simulink model "mcb_pmsm_foc_sensorless_f28069MLaunchPad"  (R2024a)
settings: Solver=FixedStepDiscrete  StartTime=0.0  StopTime=8  RelTol=1e-3  EnableMultiTasking=on
InitFcn:
  | mcb_pmsm_foc_sensorless_f28069MLaunchPad_datascript;
undefined symbols (not defined in the file): acceleration, Down, GPTRIP1SEL, GPTRIP2SEL, inverter, MAX_OL_NEG_SPD, MAX_OL_POS_SPD, MAX_OL_VD_LIMIT, MIN_CL_NEG_SPD, MIN_CL_POS_SPD, MIN_OL_VD_LIMIT, one_sec_tick, PI_params, pmsm, PU_System, RAMP_STEP_SIZE, target, Ts, Ts_motor, Ts_simulink, Ts_speed, two_sec_tick, TZ1, TZ2, Up
libraries: mcbcontrolslib x16, c2802xlib x5, simulink x4, c280xlib x4, slpidlib x3, mcbpositiondecoderlib x3, c2806xlib x3, mcbsensorlessestimatorlib x2, svdschedulerlib x2, mcbplantlib x1, autolibpmsmexterior x1
(part 2 of 3)

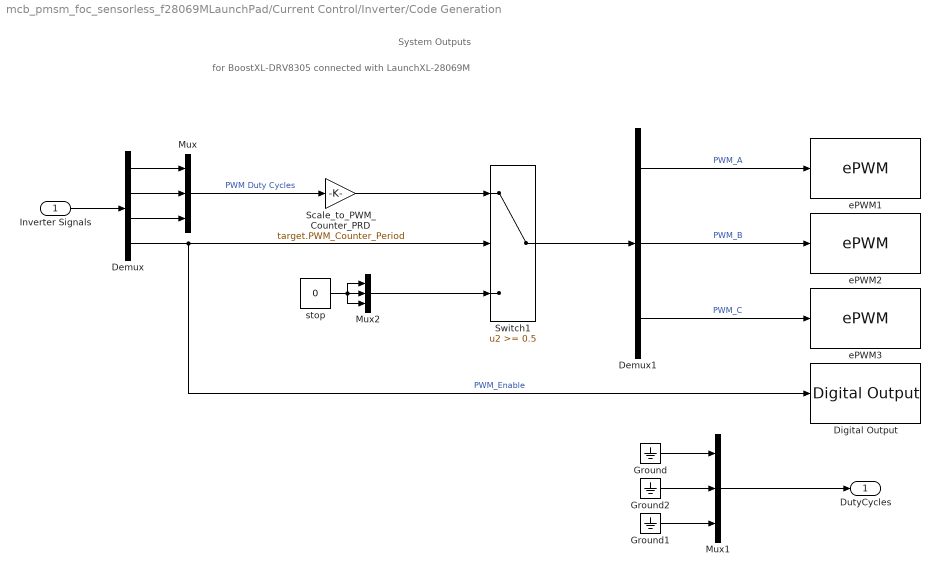
== system mcb_pmsm_foc_sensorless_f28069MLaunchPad/Current Control/Inverter/Code Generation ==
  note: for BoostXL-DRV8305 connected with LaunchXL-28069M
  note: System Outputs
  Inverter Signals : Inport
  Demux : Demux
  Demux1 : Demux  Outputs=3
  Digital Output : c2806xlib/Digital Output  GPIO_Number=GPIO50~GPIO55  GPIO_Bit0=off  GPIO_BIT0_Toggle=off  GPIO_Bit1=off  GPIO_BIT1_Toggle=off  GPIO_Bit2=on  GPIO_BIT2_Toggle=off  GPIO_Bit3=off  GPIO_BIT3_Toggle=off  GPIO_Bit4=off  GPIO_BIT4_Toggle=off  GPIO_Bit5=off  GPIO_BIT5_Toggle=off  GPIO_Bit6=off  GPIO_BIT6_Toggle=off  GPIO_Bit7=off  GPIO_BIT7_Toggle=off
  Ground : Ground
  Ground1 : Ground
  Ground2 : Ground
  Mux : Mux  Inputs=3
  Mux1 : Mux  Inputs=3
  Mux2 : Mux  Inputs=3
  Scale_to_PWM_Counter_PRD : Gain  Gain=target.PWM_Counter_Period  OutDataTypeStr=uint16  RndMeth=Simplest
  Switch1 : Switch  Threshold=0.5  SaturateOnIntegerOverflow=off  InputSameDT=off
  ePWM1 : c2802xlib/ePWM  PwmType=C2000  useModule=ePWM1  ePWMxLINKTBPRD=Not Linked  periodUnits=Clock cycles  timerSource=Specify via dialog  timerPeriod_clk=target.PWM_Counter_Period  timerPeriod_sec=64000  tbshadow=Counter equals to zero  countingMode=Up-Down  phaseActiveEnable=Disable  phaseDirection=Count down after sync  phaseActive=0  synchronizationEnable=off  dcaevt1Sync=off  dcbevt1Sync=off  synchronizationOption=Counter equals to zero (CTR=Zero)  dcbevt1SyncOut=off  dcaevt1SyncOut=off  cmpdSyncOut=off  cmpcSyncOut=off  cmpbSyncOut=off  zeroSyncOut=on  swfSyncOut=off  perSynchronizationOption=Counter equals to period (CTR=PRD)  clockPrescale=1  HSclockPrescale=1  enswap=off  ePWMxAStatus=on  ePWMxAactionLogic1=Do nothing  ePWMxAactionLogic2=Do nothing  ePWMxAactionLogic3=Clear  ePWMxAactionLogic4=Set  ePWMxAactionLogic5=Do nothing  ePWMxAactionLogic6=Do nothing  ePWMxACSFenable=off  ePWMxACSFvalue=Forcing disable  ePWMxASFreload=Zero  ePWMxBStatus=off  ePWMxBactionLogic1=Do nothing  ePWMxBactionLogic2=Set  ePWMxBactionLogic3=Do nothing  ePWMxBactionLogic4=Do nothing  ePWMxBactionLogic5=Clear  ePWMxBactionLogic6=Do nothing  ePWMxBCSFenable=off  ePWMxBCSFvalue=Forcing disable  ePWMxBSFreload=Zero  ePWNxBOutWay=off  ePWMxLINKCMPA=Not Linked  CMPAUnits=Clock cycles  CMPASource=Input port  CMPAValue_per=32000  CMPAValue_clk=floor(target.PWM_Counter_Period/2+1)  enCMPAshadow=Counter equals to zero (CTR=Zero)  ePWMxLINKCMPB=Not Linked  CMPBUnits=Clock cycles  CMPBSource=Specify via dialog  CMPBValue_per=50  CMPBValue_clk=floor(target.PWM_Counter_Period/2+1)  enCMPBshadow=Counter equals to zero (CTR=Zero)  ePWMxLINKCMPC=Not Linked  CMPCUnits=Clock cycles  CMPCSource=Specify via dialog  CMPCValue_per=50  CMPCValue_clk=32000  enCMPCshadow=Counter equals to zero (CTR=Zero)  ePWMxLINKCMPD=Not Linked  CMPDUnits=Clock cycles  CMPDSource=Specify via dialog  CMPDValue_per=50  CMPDValue_clk=32000  enCMPDshadow=Counter equals to zero (CTR=Zero)  enableDBePWMxA=on  enableDBePWMxB=on  enhalfcycle=off  DBpolarity=Active high complementary (AHC)  DBedgeDelay=Positive  DBSource_ePWMxA=ePWMxA  DBSource_ePWMxB=ePWMxA  DBPeriodUnits=Clock cycles  DBperiodSource=Specify via dialog  REDperiod=15  FEDperiod=15  REDperiod_sec=0  FEDperiod_sec=0  LoadModeDBRED=Immediate without using shadow  LoadModeDBFED=Immediate without using shadow  adcstartModuleA=on  adcrequestEventA=First event  adcstartEventA=Counter equals to period (CTR=PRD)  adcstartEventA_type2=Digital Compare Module A Event 1 start of conversion (DCAEVT1.soc)  adcstartModuleB=off  adcrequestEventB=First event  adcstartEventB=Counter equals to zero (CTR=Zero)  adcstartEventB_type2=Counter equals to zero (CTR=Zero)  intEn=off  intPrd=First event  intSel=Counter equals to zero (CTR=Zero)  intSel_type2=Counter equals to zero (CTR=Zero)  hrpe=off  enHRPWM=off  HRPWM_LoadMode=Counter equals to period (CTR=PRD)  HRPWM_CTLMode=Duty or Period control mode  HRPWM_EDGMode=Both edge  hrpeb=off  enHRPWMB=off  HRPWM_LoadModeB=Counter equals to zero (CTR=ZERO)  HRPWM_CTLModeB=Duty or Period control mode  HRPWM_EDGModeB=Both edge  enHRDBRED=off  enHRDBFED=off  enSFO=on  enautoconv=on  chopperEnable=off  chopperFrequency=1  chopperFirstwidth=1  chopperDuty=12.5%  tripZonesource=Specify via dialog  tzselOSHT1=off  tzselOSHT2=off  tzselOSHT3=off  tzselOSHT4=off  tzselOSHT5=off  tzselOSHT6=off  tzselOSHDCAEV1=off  tzselOSHDCBEV1=off  tzselCBC1=off  tzselCBC2=off  tzselCBC3=off  tzselCBC4=off  tzselCBC5=off  tzselCBC6=off  tzselCBCDCAEV2=off  tzselCBCDCBEV2=off  enTzOstIntr=off  enTzCbcIntr=off  enTzDCAEVT1Intr=off  enTzDCAEVT2Intr=off  enTzDCBEVT1Intr=off  enTzDCBEVT2Intr=off  tzclrCBCLatch=Counter equals to zero (CTR=Zero)  ePWMxAforced=No action  ePWMxBforced=No action  DCAEVT1forced=No action  DCBEVT1forced=No action  DCAEVT2forced=No action  DCBEVT2forced=No action  dcah=Trip Zone 1 input (TZ1)  dcal=Trip Zone 2 input (TZ2)  dcbh=Trip Zone 1 input (TZ1)  dcbl=Trip Zone 2 input (TZ2)  dcah_type2=GPTRIP1SEL/(TZ1)  dcal_type2=GPTRIP2SEL/(TZ2)  dcbh_type2=GPTRIP1SEL/(TZ1)  dcbl_type2=GPTRIP2SEL/(TZ2)  gendcaevt1=Event disabled  gendcaevt2=Event disabled  gendcbevt1=Event disabled  gendcbevt2=Event disabled  dcaevt1src=DCAEVT1 with sync  dcaevt2src=DCAEVT2 with sync  dcbevt1src=DCBEVT1 with sync  dcbevt2src=DCBEVT2 with sync  pulsesel=Counter equals to zero (CTR=Zero)  blankinv=off  blankoffset=0  blankwidth=0  evsrcsel=Filtered version of DCAEVT1 (DCAEVT1FILT)  encape=off
  ePWM2 : c2802xlib/ePWM  PwmType=C2000  useModule=ePWM2  ePWMxLINKTBPRD=Not Linked  periodUnits=Clock cycles  timerSource=Specify via dialog  timerPeriod_clk=target.PWM_Counter_Period  timerPeriod_sec=64000  tbshadow=Counter equals to zero  countingMode=Up-Down  phaseActiveEnable=Set counter to phase value specified via dialog  phaseDirection=Count up after sync  phaseActive=0  synchronizationEnable=off  dcaevt1Sync=off  dcbevt1Sync=off  synchronizationOption=Pass through (EPWMxSYNCI or SWFSYNC)  dcbevt1SyncOut=off  dcaevt1SyncOut=off  cmpdSyncOut=off  cmpcSyncOut=off  cmpbSyncOut=off  zeroSyncOut=off  swfSyncOut=on  perSynchronizationOption=Counter equals to period (CTR=PRD)  clockPrescale=1  HSclockPrescale=1  enswap=off  ePWMxAStatus=on  ePWMxAactionLogic1=Do nothing  ePWMxAactionLogic2=Do nothing  ePWMxAactionLogic3=Clear  ePWMxAactionLogic4=Set  ePWMxAactionLogic5=Do nothing  ePWMxAactionLogic6=Do nothing  ePWMxACSFenable=off  ePWMxACSFvalue=Forcing disable  ePWMxASFreload=Zero  ePWMxBStatus=off  ePWMxBactionLogic1=Do nothing  ePWMxBactionLogic2=Set  ePWMxBactionLogic3=Do nothing  ePWMxBactionLogic4=Do nothing  ePWMxBactionLogic5=Clear  ePWMxBactionLogic6=Do nothing  ePWMxBCSFenable=off  ePWMxBCSFvalue=Forcing disable  ePWMxBSFreload=Zero  ePWNxBOutWay=off  ePWMxLINKCMPA=Not Linked  CMPAUnits=Clock cycles  CMPASource=Input port  CMPAValue_per=32000  CMPAValue_clk=floor(target.PWM_Counter_Period/2+1)  enCMPAshadow=Counter equals to zero (CTR=Zero)  ePWMxLINKCMPB=Not Linked  CMPBUnits=Clock cycles  CMPBSource=Specify via dialog  CMPBValue_per=50  CMPBValue_clk=floor(target.PWM_Counter_Period/2+1)  enCMPBshadow=Counter equals to zero (CTR=Zero)  ePWMxLINKCMPC=Not Linked  CMPCUnits=Clock cycles  CMPCSource=Specify via dialog  CMPCValue_per=50  CMPCValue_clk=32000  enCMPCshadow=Counter equals to zero (CTR=Zero)  ePWMxLINKCMPD=Not Linked  CMPDUnits=Clock cycles  CMPDSource=Specify via dialog  CMPDValue_per=50  CMPDValue_clk=32000  enCMPDshadow=Counter equals to zero (CTR=Zero)  enableDBePWMxA=on  enableDBePWMxB=on  enhalfcycle=off  DBpolarity=Active high complementary (AHC)  DBedgeDelay=Positive  DBSource_ePWMxA=ePWMxA  DBSource_ePWMxB=ePWMxA  DBPeriodUnits=Clock cycles  DBperiodSource=Specify via dialog  REDperiod=15  FEDperiod=15  REDperiod_sec=0  FEDperiod_sec=0  LoadModeDBRED=Immediate without using shadow  LoadModeDBFED=Immediate without using shadow  adcstartModuleA=off  adcrequestEventA=First event  adcstartEventA=Digital Compare Module A Event 1 start of conversion (DCAEVT1.soc)  adcstartEventA_type2=Digital Compare Module A Event 1 start of conversion (DCAEVT1.soc)  adcstartModuleB=off  adcrequestEventB=First event  adcstartEventB=Counter equals to zero (CTR=Zero)  adcstartEventB_type2=Counter equals to zero (CTR=Zero)  intEn=off  intPrd=First event  intSel=Counter equals to zero (CTR=Zero)  intSel_type2=Counter equals to zero (CTR=Zero)  hrpe=off  enHRPWM=off  HRPWM_LoadMode=Counter equals to period (CTR=PRD)  HRPWM_CTLMode=Duty or Period control mode  HRPWM_EDGMode=Both edge  hrpeb=off  enHRPWMB=off  HRPWM_LoadModeB=Counter equals to zero (CTR=ZERO)  HRPWM_CTLModeB=Duty or Period control mode  HRPWM_EDGModeB=Both edge  enHRDBRED=off  enHRDBFED=off  enSFO=on  enautoconv=on  chopperEnable=off  chopperFrequency=1  chopperFirstwidth=1  chopperDuty=12.5%  tripZonesource=Specify via dialog  tzselOSHT1=off  tzselOSHT2=off  tzselOSHT3=off  tzselOSHT4=off  tzselOSHT5=off  tzselOSHT6=off  tzselOSHDCAEV1=off  tzselOSHDCBEV1=off  tzselCBC1=off  tzselCBC2=off  tzselCBC3=off  tzselCBC4=off  tzselCBC5=off  tzselCBC6=off  tzselCBCDCAEV2=off  tzselCBCDCBEV2=off  enTzOstIntr=off  enTzCbcIntr=off  enTzDCAEVT1Intr=off  enTzDCAEVT2Intr=off  enTzDCBEVT1Intr=off  enTzDCBEVT2Intr=off  tzclrCBCLatch=Counter equals to zero (CTR=Zero)  ePWMxAforced=No action  ePWMxBforced=No action  DCAEVT1forced=No action  DCBEVT1forced=No action  DCAEVT2forced=No action  DCBEVT2forced=No action  dcah=Trip Zone 1 input (TZ1)  dcal=Trip Zone 2 input (TZ2)  dcbh=Trip Zone 1 input (TZ1)  dcbl=Trip Zone 2 input (TZ2)  dcah_type2=GPTRIP1SEL/(TZ1)  dcal_type2=GPTRIP2SEL/(TZ2)  dcbh_type2=GPTRIP1SEL/(TZ1)  dcbl_type2=GPTRIP2SEL/(TZ2)  gendcaevt1=Event disabled  gendcaevt2=Event disabled  gendcbevt1=Event disabled  gendcbevt2=Event disabled  dcaevt1src=DCAEVT1 with sync  dcaevt2src=DCAEVT2 with sync  dcbevt1src=DCBEVT1 with sync  dcbevt2src=DCBEVT2 with sync  pulsesel=Counter equals to zero (CTR=Zero)  blankinv=off  blankoffset=0  blankwidth=0  evsrcsel=Filtered version of DCAEVT1 (DCAEVT1FILT)  encape=off
  ePWM3 : c2802xlib/ePWM  PwmType=C2000  useModule=ePWM3  ePWMxLINKTBPRD=Not Linked  periodUnits=Clock cycles  timerSource=Specify via dialog  timerPeriod_clk=target.PWM_Counter_Period  timerPeriod_sec=64000  tbshadow=Counter equals to zero  countingMode=Up-Down  phaseActiveEnable=Set counter to phase value specified via dialog  phaseDirection=Count up after sync  phaseActive=0  synchronizationEnable=off  dcaevt1Sync=off  dcbevt1Sync=off  synchronizationOption=Disable  dcbevt1SyncOut=off  dcaevt1SyncOut=off  cmpdSyncOut=off  cmpcSyncOut=off  cmpbSyncOut=off  zeroSyncOut=off  swfSyncOut=off  perSynchronizationOption=Counter equals to period (CTR=PRD)  clockPrescale=1  HSclockPrescale=1  enswap=off  ePWMxAStatus=on  ePWMxAactionLogic1=Do nothing  ePWMxAactionLogic2=Do nothing  ePWMxAactionLogic3=Clear  ePWMxAactionLogic4=Set  ePWMxAactionLogic5=Do nothing  ePWMxAactionLogic6=Do nothing  ePWMxACSFenable=off  ePWMxACSFvalue=Forcing disable  ePWMxASFreload=Zero  ePWMxBStatus=off  ePWMxBactionLogic1=Do nothing  ePWMxBactionLogic2=Set  ePWMxBactionLogic3=Do nothing  ePWMxBactionLogic4=Do nothing  ePWMxBactionLogic5=Clear  ePWMxBactionLogic6=Do nothing  ePWMxBCSFenable=off  ePWMxBCSFvalue=Forcing disable  ePWMxBSFreload=Zero  ePWNxBOutWay=off  ePWMxLINKCMPA=Not Linked  CMPAUnits=Clock cycles  CMPASource=Input port  CMPAValue_per=32000  CMPAValue_clk=floor(target.PWM_Counter_Period/2+1)  enCMPAshadow=Counter equals to zero (CTR=Zero)  ePWMxLINKCMPB=Not Linked  CMPBUnits=Clock cycles  CMPBSource=Specify via dialog  CMPBValue_per=50  CMPBValue_clk=floor(target.PWM_Counter_Period/2+1)  enCMPBshadow=Counter equals to zero (CTR=Zero)  ePWMxLINKCMPC=Not Linked  CMPCUnits=Clock cycles  CMPCSource=Specify via dialog  CMPCValue_per=50  CMPCValue_clk=32000  enCMPCshadow=Counter equals to zero (CTR=Zero)  ePWMxLINKCMPD=Not Linked  CMPDUnits=Clock cycles  CMPDSource=Specify via dialog  CMPDValue_per=50  CMPDValue_clk=32000  enCMPDshadow=Counter equals to zero (CTR=Zero)  enableDBePWMxA=on  enableDBePWMxB=on  enhalfcycle=off  DBpolarity=Active high complementary (AHC)  DBedgeDelay=Positive  DBSource_ePWMxA=ePWMxA  DBSource_ePWMxB=ePWMxA  DBPeriodUnits=Clock cycles  DBperiodSource=Specify via dialog  REDperiod=15  FEDperiod=15  REDperiod_sec=0  FEDperiod_sec=0  LoadModeDBRED=Immediate without using shadow  LoadModeDBFED=Immediate without using shadow  adcstartModuleA=off  adcrequestEventA=First event  adcstartEventA=Digital Compare Module A Event 1 start of conversion (DCAEVT1.soc)  adcstartEventA_type2=Digital Compare Module A Event 1 start of conversion (DCAEVT1.soc)  adcstartModuleB=off  adcrequestEventB=First event  adcstartEventB=Counter equals to zero (CTR=Zero)  adcstartEventB_type2=Counter equals to zero (CTR=Zero)  intEn=off  intPrd=First event  intSel=Counter equals to zero (CTR=Zero)  intSel_type2=Counter equals to zero (CTR=Zero)  hrpe=off  enHRPWM=off  HRPWM_LoadMode=Counter equals to period (CTR=PRD)  HRPWM_CTLMode=Duty or Period control mode  HRPWM_EDGMode=Both edge  hrpeb=off  enHRPWMB=off  HRPWM_LoadModeB=Counter equals to zero (CTR=ZERO)  HRPWM_CTLModeB=Duty or Period control mode  HRPWM_EDGModeB=Both edge  enHRDBRED=off  enHRDBFED=off  enSFO=on  enautoconv=on  chopperEnable=off  chopperFrequency=1  chopperFirstwidth=1  chopperDuty=12.5%  tripZonesource=Specify via dialog  tzselOSHT1=off  tzselOSHT2=off  tzselOSHT3=off  tzselOSHT4=off  tzselOSHT5=off  tzselOSHT6=off  tzselOSHDCAEV1=off  tzselOSHDCBEV1=off  tzselCBC1=off  tzselCBC2=off  tzselCBC3=off  tzselCBC4=off  tzselCBC5=off  tzselCBC6=off  tzselCBCDCAEV2=off  tzselCBCDCBEV2=off  enTzOstIntr=off  enTzCbcIntr=off  enTzDCAEVT1Intr=off  enTzDCAEVT2Intr=off  enTzDCBEVT1Intr=off  enTzDCBEVT2Intr=off  tzclrCBCLatch=Counter equals to zero (CTR=Zero)  ePWMxAforced=No action  ePWMxBforced=No action  DCAEVT1forced=No action  DCBEVT1forced=No action  DCAEVT2forced=No action  DCBEVT2forced=No action  dcah=Trip Zone 1 input (TZ1)  dcal=Trip Zone 2 input (TZ2)  dcbh=Trip Zone 1 input (TZ1)  dcbl=Trip Zone 2 input (TZ2)  dcah_type2=GPTRIP1SEL/(TZ1)  dcal_type2=GPTRIP2SEL/(TZ2)  dcbh_type2=GPTRIP1SEL/(TZ1)  dcbl_type2=GPTRIP2SEL/(TZ2)  gendcaevt1=Event disabled  gendcaevt2=Event disabled  gendcbevt1=Event disabled  gendcbevt2=Event disabled  dcaevt1src=DCAEVT1 with sync  dcaevt2src=DCAEVT2 with sync  dcbevt1src=DCBEVT1 with sync  dcbevt2src=DCBEVT2 with sync  pulsesel=Counter equals to zero (CTR=Zero)  blankinv=off  blankoffset=0  blankwidth=0  evsrcsel=Filtered version of DCAEVT1 (DCAEVT1FILT)  encape=off
  stop : Constant  Value=0  OutDataTypeStr=uint16
  DutyCycles : Outport  VectorParamsAs1DForOutWhenUnconnected=off
  wires:
  Demux1/3 -> ePWM3/1  "PWM_C"
  Scale_to_PWM_Counter_PRD/1 -> Switch1/1
  Mux2/1 -> Switch1/3
  stop/1 -> Mux2/3, Mux2/2, Mux2/1
  Demux/4 -> Switch1/2, Digital Output/1  "PWM_Enable"
  Inverter Signals/1 -> Demux/1
  Demux1/2 -> ePWM2/1  "PWM_B"
  Switch1/1 -> Demux1/1
  Demux1/1 -> ePWM1/1  "PWM_A"
  Mux/1 -> Scale_to_PWM_Counter_PRD/1  "PWM Duty Cycles"
  Ground/1 -> Mux1/1
  Ground1/1 -> Mux1/3
  Ground2/1 -> Mux1/2
  Mux1/1 -> DutyCycles/1
  Demux/1 -> Mux/1
  Demux/2 -> Mux/2
  Demux/3 -> Mux/3

== system mcb_pmsm_foc_sensorless_f28069MLaunchPad/Current Control/Inverter/Simulation ==
  Inverter Signals : Inport
  Data Type Duplicate : DataTypeDuplicate
  Demux : Demux
  Mux : Mux  Inputs=3
  Mux2 : Mux  Inputs=3
  Switch1 : Switch  Threshold=0.5  RndMeth=Simplest  SaturateOnIntegerOverflow=off  InputSameDT=off
  stop : Constant  Value=0  OutDataTypeStr=Inherit: Inherit via back propagation
  DutyCycles : Outport  VectorParamsAs1DForOutWhenUnconnected=off
  wires:
  stop/1 -> Data Type Duplicate/2, Mux2/1, Mux2/3, Mux2/2
  Mux2/1 -> Switch1/3
  Switch1/1 -> DutyCycles/1
  Inverter Signals/1 -> Demux/1
  Demux/4 -> Switch1/2  "PWM Enable"
  Mux/1 -> Data Type Duplicate/1, Switch1/1  "PWM Duty Cycles"
  Demux/1 -> Mux/1
  Demux/2 -> Mux/2
  Demux/3 -> Mux/3

== system mcb_pmsm_foc_sensorless_f28069MLaunchPad/Current Control/SCI_Tx/Code Generation ==
  SCI_Data : Inport
  CodeGeneration : Subsystem  TreatAsAtomicUnit=on
  wires:
  SCI_Data/1 -> CodeGeneration/1(Input)

== system mcb_pmsm_foc_sensorless_f28069MLaunchPad/Current Control/SCI_Tx/Simulation ==
  SCI_Data : Inport
  Demux : Demux  Outputs=2
  Terminator1 : Terminator
  Terminator2 : Terminator
  wires:
  SCI_Data/1 -> Demux/1
  Demux/1 -> Terminator1/1
  Demux/2 -> Terminator2/1

== system mcb_pmsm_foc_sensorless_f28069MLaunchPad/Hardware Init/Variant Subsystem/Code Generation ==
  note: for BoostXL-DRV8305 connected to LaunchXL-28069M
  note: System Outputs
  In1 : Inport
  ADC Calib Enable : Constant  Value=inverter.ADCOffsetCalibEnable
  "Calculate ADC Offset " : Subsystem  Priority=1001  TreatAsAtomicUnit=on
  DRV Enable : Subsystem  Priority=1
  Default ADC Offset : Subsystem  Priority=1001  TreatAsAtomicUnit=on
  NOT : Logic  Operator=NOT  IconShape=distinctive  AllPortsSameDT=off  OutDataTypeStr=boolean
  wires:
  In1/1 -> DRV Enable/1(In)
  NOT/1 -> Default ADC Offset/Enable
  ADC Calib Enable/1 -> "Calculate ADC Offset "/Enable, NOT/1

== system mcb_pmsm_foc_sensorless_f28069MLaunchPad/Hardware Init/Variant Subsystem/Simulation ==
  In1 : Inport
  Terminator : Terminator
  wires:
  In1/1 -> Terminator/1

== system mcb_pmsm_foc_sensorless_f28069MLaunchPad/Heartbeat LED/Heartbeat LED/Code generation ==
  In1 : Inport
  Digital Output1 : c2806xlib/Digital Output  GPIO_Number=GPIO32~GPIO39  GPIO_Bit0=off  GPIO_BIT0_Toggle=off  GPIO_Bit1=off  GPIO_BIT1_Toggle=off  GPIO_Bit2=on  GPIO_BIT2_Toggle=on  GPIO_Bit3=off  GPIO_BIT3_Toggle=off  GPIO_Bit4=off  GPIO_BIT4_Toggle=off  GPIO_Bit5=off  GPIO_BIT5_Toggle=off  GPIO_Bit6=off  GPIO_BIT6_Toggle=off  GPIO_Bit7=off  GPIO_BIT7_Toggle=off
  wires:
  In1/1 -> Digital Output1/1

== system mcb_pmsm_foc_sensorless_f28069MLaunchPad/Heartbeat LED/Heartbeat LED/Simulation ==
  In1 : Inport
  Simulation_Terminator : Terminator
  wires:
  In1/1 -> Simulation_Terminator/1

== system mcb_pmsm_foc_sensorless_f28069MLaunchPad/Inverter and Motor - Plant Model/Simulation/Inverter ==
  Duty_abc : Inport
  Average-Value Inverter : mcbplantlib/Average-Value Inverter
  Constant2 : Constant  Value=inverter.V_dc  OutDataTypeStr=single  SampleTime=-1
  Data Type Conversion1 : DataTypeConversion  OutDataTypeStr=single  RndMeth=Simplest  SaturateOnIntegerOverflow=off
  Rate Transition3 : RateTransition  Deterministic=off  OutPortSampleTime=Ts_inverter
  Vabc : Outport  VectorParamsAs1DForOutWhenUnconnected=off
  wires:
  Constant2/1 -> Average-Value Inverter/2
  Data Type Conversion1/1 -> Rate Transition3/1
  Duty_abc/1 -> Data Type Conversion1/1
  Average-Value Inverter/1 -> Vabc/1
  Rate Transition3/1 -> Average-Value Inverter/1

== system mcb_pmsm_foc_sensorless_f28069MLaunchPad/Inverter and Motor - Plant Model/Simulation/Load_Profile (Torque) ==
  Data Type Conversion : DataTypeConversion  OutDataTypeStr=single  SaturateOnIntegerOverflow=off  RndMeth=Floor
  IIR Filter : mcbcontrolslib/IIR Filter  VariantControl=Low Pass Filter  VariantSelect=Low-pass  FilterConstantInputType=Specify via dialog  Filter_constant=0.0001  advancedSettings=off  Ts=50e-6  cutOff_freq=0.31834
  T_load : Step  Time=4  Before=0.05*pmsm.T_rated  After=0.05*pmsm.T_rated  SampleTime=Ts_simulink
  Load_Trq : Outport  VectorParamsAs1DForOutWhenUnconnected=off
  wires:
  Data Type Conversion/1 -> IIR Filter/1
  IIR Filter/1 -> Load_Trq/1
  T_load/1 -> Data Type Conversion/1

== system mcb_pmsm_foc_sensorless_f28069MLaunchPad/Inverter and Motor - Plant Model/Simulation/Sensor_Measurements ==
  note: Scaling
  note: Delays
  PhaseCurr : Inport
  Add Offset : Sum  RndMeth=Simplest
  Data Type Conversion4 : DataTypeConversion  OutDataTypeStr=single  RndMeth=Simplest  SaturateOnIntegerOverflow=off
  Delay1 : Delay  DelayLength=PI_params.delay_Currents
  Get ADC Count : Gain  Gain=target.ADC_MaxCount/target.ADC_Vref  OutMin=0  OutMax=target.ADC_MaxCount  OutDataTypeStr=uint16  RndMeth=Simplest
  Get Current Sense Voltage : Gain  Gain=inverter.invertingAmp * inverter.ISenseVoltPerAmp  RndMeth=Simplest  OutDataTypeStr=Inherit: Same as input
  Offset voltage : Gain  Gain=target.ADC_Vref / target.ADC_MaxCount  RndMeth=Simplest
  Saturate at ADC Vref : Saturate  UpperLimit=target.ADC_Vref  LowerLimit=0
  Saturate at inverter Vref : Saturate  UpperLimit=inverter.ISenseVref  LowerLimit=0
  Selector : Selector  InputPortWidth=3  IndexOptions=Index vector (dialog)  Indices=[1 2]  OutputSizes=1
  ~1.65V in ADC counts : Constant  Value=[inverter.CtSensAOffset inverter.CtSensBOffset]  OutDataTypeStr=uint16  SampleTime=-1
  Sim_fb : Outport  VectorParamsAs1DForOutWhenUnconnected=off
  wires:
  Delay1/1 -> Selector/1  "Iab_fb"
  Data Type Conversion4/1 -> Delay1/1
  PhaseCurr/1 -> Data Type Conversion4/1
  Add Offset/1 -> Saturate at inverter Vref/1
  Saturate at inverter Vref/1 -> Saturate at ADC Vref/1
  ~1.65V in ADC counts/1 -> Offset voltage/1
  Get Current Sense Voltage/1 -> Add Offset/1
  Saturate at ADC Vref/1 -> Get ADC Count/1
  Selector/1 -> Get Current Sense Voltage/1
  Offset voltage/1 -> Add Offset/2
  Get ADC Count/1 -> Sim_fb/1

== system mcb_pmsm_foc_sensorless_f28069MLaunchPad/Serial Receive/SCI_Rx/Code Generation ==
  SCI Receive : c280xlib/SCI Receive  sciModule=A  dataHead=''  headerCheckMaxCount=16  dataTail=''  dataType=uint16  dataLenOptions=Length via dialog  dataDim=2  maxDataLength=1  initValue=0  errOption=Output the last received value  errValue=0  sampleTime=-1  blockingMode=on  timeOut=0.019444  outputStatus=off
  Data : Outport
  wires:
  SCI Receive/1 -> Data/1

== system mcb_pmsm_foc_sensorless_f28069MLaunchPad/Serial Receive/SCI_Rx/Simulation ==
  Data Type Conversion : DataTypeConversion  OutDataTypeStr=fixdt(1,16,12)  RndMeth=Simplest  SaturateOnIntegerOverflow=off
  Data Type Conversion2 : DataTypeConversion  OutDataTypeStr=single  RndMeth=Simplest  SaturateOnIntegerOverflow=off
  Data Type Conversion3 : DataTypeConversion  OutDataTypeStr=uint32  ConvertRealWorld=Stored Integer (SI)  RndMeth=Simplest  SaturateOnIntegerOverflow=off
  Data Type Conversion4 : DataTypeConversion  OutDataTypeStr=single  RndMeth=Simplest  SaturateOnIntegerOverflow=off
  Enable : Constant  OutDataTypeStr=dataType  SampleTime=-1
  Mux : Mux  Inputs=2
  Speed_Ref_CW (rpm) : Step  Time=4  Before=0.6*pmsm.N_base  After=-0.6*pmsm.N_base
  rpm2PU : Gain  Gain=1/pmsm.N_base  RndMeth=Simplest  OutDataTypeStr=Inherit: Same as input
  Data : Outport
  wires:
  rpm2PU/1 -> Data Type Conversion2/1
  Enable/1 -> Data Type Conversion4/1
  Data Type Conversion2/1 -> Mux/1
  Data Type Conversion4/1 -> Mux/2
  Mux/1 -> Data Type Conversion/1
  Data Type Conversion/1 -> Data Type Conversion3/1
  Data Type Conversion3/1 -> Data/1
  Speed_Ref_CW (rpm)/1 -> rpm2PU/1

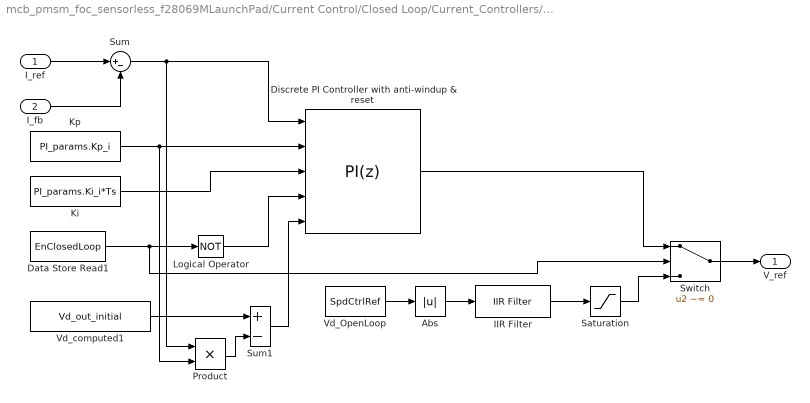
== system mcb_pmsm_foc_sensorless_f28069MLaunchPad/Current Control/Closed Loop/Current_Controllers/PI_Controller_Id ==
  I_ref : Inport
  I_fb : Inport  Port=2
  Abs : Abs  RndMeth=Simplest  SaturateOnIntegerOverflow=off
  Data Store Read1 : DataStoreRead  DataStoreName=EnClosedLoop  IndexOptions=Index vector (dialog)  Indices=1  OutputSizes=1
  Discrete PI Controller with anti-windup & reset : slpidlib/PID Controller  Controller=PI  Form=Parallel  TimeDomain=Discrete-time  UseExternalTs=off  SampleTime=-1  IntegratorMethod=Forward Euler  FilterMethod=Forward Euler  ControllerParametersSource=external  P=1  I=1  UseKiTs=on  D=0  UseExternalDerivativeSource=off  N=100  UseFilter=on  TunerSelectOption=Transfer Function Based (PID Tuner App)  InitialConditionSource=external  InitialConditionForIntegrator=0  InitialConditionForFilter=0  DifferentiatorICPrevScaledInput=0  ExternalReset=level  TrackingMode=off  Kt=1  LimitOutput=on  SatLimitsSource=internal  UpperSaturationLimit=1  LowerSaturationLimit=-1  LinearizeAsGain=on  AntiWindupMode=clamping  Kb=1  LimitIntegrator=off  UpperIntegratorSaturationLimit=inf  LowerIntegratorSaturationLimit=-inf  RndMeth=Simplest  POutMin=[]  POutMax=[]  IOutMin=[]  IOutMax=[]  DOutMin=[]  DOutMax=[]  NOutMin=[]  NOutMax=[]  SumOutMin=[]  SumOutMax=[]  SaturationOutDataTypeStr=Inherit: Inherit via back propagation  SaturationOutMin=[]  SaturationOutMax=[]  PParamMin=[]  PParamMax=[]  IParamMin=[]  IParamMax=[]  DParamMin=[]  DParamMax=[]  NParamMin=[]  NParamMax=[]  KbParamMin=[]  KbParamMax=[]  KtParamMin=[]  KtParamMax=[]  KbOutMin=[]  KbOutMax=[]  KtOutMin=[]  KtOutMax=[]  IntegratorOutMin=[]  IntegratorOutMax=[]  FilterOutMin=[]  FilterOutMax=[]  SumI1OutMin=[]  SumI1OutMax=[]  SumI2OutMin=[]  SumI2OutMax=[]  SumI3OutMin=[]  SumI3OutMax=[]  SumI4OutMin=[]  SumI4OutMax=[]  SumDOutMin=[]  SumDOutMax=[]  DifferentiatorOutMin=[]  DifferentiatorOutMax=[]  FilterDiffOutCoefMin=[]  FilterDiffOutCoefMax=[]  ReciprocalOutMin=[]  ReciprocalOutMax=[]  SumDenOutMin=[]  SumDenOutMax=[]  SumNumOutMin=[]  SumNumOutMax=[]  DivideOutMin=[]  DivideOutMax=[]  UdiffTsProdOutMin=[]  UdiffTsProdOutMax=[]  NTsProdOutMin=[]  NTsProdOutMax=[]  UintegralTsProdOutMin=[]  UintegralTsProdOutMax=[]  UngainTsProdOutMin=[]  UngainTsProdOutMax=[]  ClampingZeroOutDataTypeStr=Inherit: Inherit via back propagation  ClampingZeroOutMin=[]  ClampingZeroOutMax=[]  FilterDenConstantOutDataTypeStr=Inherit: Inherit via back propagation  FilterDenConstantOutMin=[]  FilterDenConstantOutMax=[]  PCopyOutDataTypeStr=Inherit: Inherit via back propagation  PCopyOutMin=[]  PCopyOutMax=[]  NCopyOutDataTypeStr=Inherit: Inherit via back propagation  NCopyOutMin=[]  NCopyOutMax=[]  IntegratorContinuousStateAttributes=''  IntegratorStateMustResolveToSignalObject=off  IntegratorRTWStateStorageClass=Auto  FilterContinuousStateAttributes=''  FilterStateMustResolveToSignalObject=off  FilterRTWStateStorageClass=Auto  ParallelPVariant=ExternalParameters  IdealPVariant=Disabled  IVariant=ExternalParameters  DVariant=Disabled  IntegratorVariant=Discrete  SatVariant=Enabled  AWVariant=DiscClampingParallel  PCopyVariant=Disabled  TRVariant=Disabled  FdbkBlocksVariant=Forward  IdealPFdbkVariant=Disabled  SatFdbkVariant=Disabled  DerivativeFilterVariant=Disabled  NVariant=Disabled  NCopyVariant=Disabled_SignalSpec  FilterICVariant=Disabled  IntegratorICVariant=ExternalICs  ExternalResetVariant=ExternalReset  TRSumVariant=Passthrough  SumFdbkVariant=Disabled  SumVariant=Sum_PI  TsampFilterVariant=InternalTs  TsampNgainVariant=Passthrough  TsampIntegralVariant=Disabled_SignalSpec  ExternalSaturationOutDataTypeStr=Inherit: Same as second input  DerivativeSourceVariant=Disabled
      settings: LibrarySourceBlock=mcbcontrolslib/PI Controller
  IIR Filter : mcbcontrolslib/IIR Filter  VariantControl=Low Pass Filter  VariantSelect=Low-pass  FilterConstantInputType=Specify via dialog  Filter_constant=0.1  advancedSettings=on  Ts=50e-6  cutOff_freq=353.6777
      settings: LibrarySourceBlock=mcblib/Signal Management/IIR Filter
  Ki : Constant  Value=PI_params.Ki_i*Ts  OutDataTypeStr=dataType  SampleTime=-1
  Kp : Constant  Value=PI_params.Kp_i  OutDataTypeStr=dataType  SampleTime=-1
  Logical Operator : Logic  Operator=NOT  IconShape=distinctive  AllPortsSameDT=off  OutDataTypeStr=boolean
  Product : Product  RndMeth=Simplest  OutDataTypeStr=Inherit: Same as first input
  Saturation : Saturate  UpperLimit=MAX_OL_VD_LIMIT  LowerLimit=MIN_OL_VD_LIMIT  RndMeth=Simplest
  Sum : Sum  Inputs=|+-  OutDataTypeStr=Inherit: Same as first input
  Sum1 : Sum  Inputs=+-  RndMeth=Simplest  OutDataTypeStr=Inherit: Same as first input
  Switch : Switch  Criteria=u2 ~= 0  RndMeth=Simplest  SaturateOnIntegerOverflow=off  InputSameDT=off
  Vd_OpenLoop : DataStoreRead  DataStoreName=SpdCtrlRef  IndexOptions=Index vector (dialog)  Indices=1  OutputSizes=1
  Vd_computed1 : DataStoreRead  DataStoreName=Vd_out_initial  IndexOptions=Index vector (dialog)  Indices=1  OutputSizes=1
  V_ref : Outport  VectorParamsAs1DForOutWhenUnconnected=off
  wires:
  Switch/1 -> V_ref/1
  I_fb/1 -> Sum/2
  Sum/1 -> Product/1, Discrete PI Controller with anti-windup & reset/1
  Kp/1 -> Product/2, Discrete PI Controller with anti-windup & reset/2
  I_ref/1 -> Sum/1
  Ki/1 -> Discrete PI Controller with anti-windup & reset/3
  Logical Operator/1 -> Discrete PI Controller with anti-windup & reset/4
  Discrete PI Controller with anti-windup & reset/1 -> Switch/1
  Data Store Read1/1 -> Logical Operator/1, Switch/2
  Saturation/1 -> Switch/3
  Vd_OpenLoop/1 -> Abs/1
  Abs/1 -> IIR Filter/1
  IIR Filter/1 -> Saturation/1
  Vd_computed1/1 -> Sum1/1
  Product/1 -> Sum1/2
  Sum1/1 -> Discrete PI Controller with anti-windup & reset/5

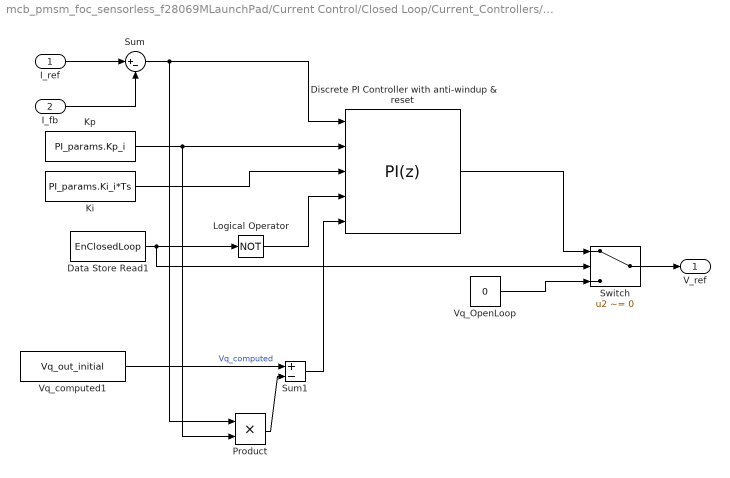
== system mcb_pmsm_foc_sensorless_f28069MLaunchPad/Current Control/Closed Loop/Current_Controllers/PI_Controller_Iq ==
  I_ref : Inport
  I_fb : Inport  Port=2
  Data Store Read1 : DataStoreRead  DataStoreName=EnClosedLoop  IndexOptions=Index vector (dialog)  Indices=1  OutputSizes=1
  Discrete PI Controller with anti-windup & reset : slpidlib/PID Controller  Controller=PI  Form=Parallel  TimeDomain=Discrete-time  UseExternalTs=off  SampleTime=-1  IntegratorMethod=Forward Euler  FilterMethod=Forward Euler  ControllerParametersSource=external  P=1  I=1  UseKiTs=on  D=0  UseExternalDerivativeSource=off  N=100  UseFilter=on  TunerSelectOption=Transfer Function Based (PID Tuner App)  InitialConditionSource=external  InitialConditionForIntegrator=0  InitialConditionForFilter=0  DifferentiatorICPrevScaledInput=0  ExternalReset=level  TrackingMode=off  Kt=1  LimitOutput=on  SatLimitsSource=internal  UpperSaturationLimit=1  LowerSaturationLimit=-1  LinearizeAsGain=on  AntiWindupMode=clamping  Kb=1  LimitIntegrator=off  UpperIntegratorSaturationLimit=inf  LowerIntegratorSaturationLimit=-inf  RndMeth=Simplest  POutMin=[]  POutMax=[]  IOutMin=[]  IOutMax=[]  DOutMin=[]  DOutMax=[]  NOutMin=[]  NOutMax=[]  SumOutMin=[]  SumOutMax=[]  SaturationOutDataTypeStr=Inherit: Inherit via back propagation  SaturationOutMin=[]  SaturationOutMax=[]  PParamMin=[]  PParamMax=[]  IParamMin=[]  IParamMax=[]  DParamMin=[]  DParamMax=[]  NParamMin=[]  NParamMax=[]  KbParamMin=[]  KbParamMax=[]  KtParamMin=[]  KtParamMax=[]  KbOutMin=[]  KbOutMax=[]  KtOutMin=[]  KtOutMax=[]  IntegratorOutMin=[]  IntegratorOutMax=[]  FilterOutMin=[]  FilterOutMax=[]  SumI1OutMin=[]  SumI1OutMax=[]  SumI2OutMin=[]  SumI2OutMax=[]  SumI3OutMin=[]  SumI3OutMax=[]  SumI4OutMin=[]  SumI4OutMax=[]  SumDOutMin=[]  SumDOutMax=[]  DifferentiatorOutMin=[]  DifferentiatorOutMax=[]  FilterDiffOutCoefMin=[]  FilterDiffOutCoefMax=[]  ReciprocalOutMin=[]  ReciprocalOutMax=[]  SumDenOutMin=[]  SumDenOutMax=[]  SumNumOutMin=[]  SumNumOutMax=[]  DivideOutMin=[]  DivideOutMax=[]  UdiffTsProdOutMin=[]  UdiffTsProdOutMax=[]  NTsProdOutMin=[]  NTsProdOutMax=[]  UintegralTsProdOutMin=[]  UintegralTsProdOutMax=[]  UngainTsProdOutMin=[]  UngainTsProdOutMax=[]  ClampingZeroOutDataTypeStr=Inherit: Inherit via back propagation  ClampingZeroOutMin=[]  ClampingZeroOutMax=[]  FilterDenConstantOutDataTypeStr=Inherit: Inherit via back propagation  FilterDenConstantOutMin=[]  FilterDenConstantOutMax=[]  PCopyOutDataTypeStr=Inherit: Inherit via back propagation  PCopyOutMin=[]  PCopyOutMax=[]  NCopyOutDataTypeStr=Inherit: Inherit via back propagation  NCopyOutMin=[]  NCopyOutMax=[]  IntegratorContinuousStateAttributes=''  IntegratorStateMustResolveToSignalObject=off  IntegratorRTWStateStorageClass=Auto  FilterContinuousStateAttributes=''  FilterStateMustResolveToSignalObject=off  FilterRTWStateStorageClass=Auto  ParallelPVariant=ExternalParameters  IdealPVariant=Disabled  IVariant=ExternalParameters  DVariant=Disabled  IntegratorVariant=Discrete  SatVariant=Enabled  AWVariant=DiscClampingParallel  PCopyVariant=Disabled  TRVariant=Disabled  FdbkBlocksVariant=Forward  IdealPFdbkVariant=Disabled  SatFdbkVariant=Disabled  DerivativeFilterVariant=Disabled  NVariant=Disabled  NCopyVariant=Disabled_SignalSpec  FilterICVariant=Disabled  IntegratorICVariant=ExternalICs  ExternalResetVariant=ExternalReset  TRSumVariant=Passthrough  SumFdbkVariant=Disabled  SumVariant=Sum_PI  TsampFilterVariant=InternalTs  TsampNgainVariant=Passthrough  TsampIntegralVariant=Disabled_SignalSpec  ExternalSaturationOutDataTypeStr=Inherit: Same as second input  DerivativeSourceVariant=Disabled
      settings: LibrarySourceBlock=mcbcontrolslib/PI Controller
  Ki : Constant  Value=PI_params.Ki_i*Ts  OutDataTypeStr=dataType  SampleTime=-1
  Kp : Constant  Value=PI_params.Kp_i  OutDataTypeStr=dataType  SampleTime=-1
  Logical Operator : Logic  Operator=NOT  IconShape=distinctive  AllPortsSameDT=off  OutDataTypeStr=boolean
  Product : Product  RndMeth=Simplest  OutDataTypeStr=Inherit: Same as first input
  Sum : Sum  Inputs=|+-  OutDataTypeStr=Inherit: Same as first input
  Sum1 : Sum  Inputs=+-  RndMeth=Simplest  OutDataTypeStr=Inherit: Same as first input
  Switch : Switch  Criteria=u2 ~= 0  RndMeth=Simplest  SaturateOnIntegerOverflow=off  InputSameDT=off
  Vq_OpenLoop : Constant  Value=0  OutDataTypeStr=dataType  SampleTime=-1
  Vq_computed1 : DataStoreRead  DataStoreName=Vq_out_initial  IndexOptions=Index vector (dialog)  Indices=1  OutputSizes=1
  V_ref : Outport  VectorParamsAs1DForOutWhenUnconnected=off
  wires:
  Switch/1 -> V_ref/1
  I_fb/1 -> Sum/2
  Sum/1 -> Product/1, Discrete PI Controller with anti-windup & reset/1
  Kp/1 -> Product/2, Discrete PI Controller with anti-windup & reset/2
  I_ref/1 -> Sum/1
  Ki/1 -> Discrete PI Controller with anti-windup & reset/3
  Logical Operator/1 -> Discrete PI Controller with anti-windup & reset/4
  Discrete PI Controller with anti-windup & reset/1 -> Switch/1
  Vq_OpenLoop/1 -> Switch/3
  Data Store Read1/1 -> Switch/2, Logical Operator/1
  Product/1 -> Sum1/2
  Sum1/1 -> Discrete PI Controller with anti-windup & reset/5
  Vq_computed1/1 -> Sum1/1  "Vq_computed"

== system mcb_pmsm_foc_sensorless_f28069MLaunchPad/Current Control/Closed Loop/Open_Loop_Control/Accumulate1 ==
  Theta : Inport
  Theta_e_prev : Inport  Port=2
  Add : Sum  RndMeth=Simplest  OutDataTypeStr=Inherit: Same as first input
  Add1 : Sum  Inputs=+-  OutDataTypeStr=Inherit: Inherit via back propagation  RndMeth=Simplest
  Constant : Constant  OutDataTypeStr=boolean  SampleTime=-1
  Data Type Conversion : DataTypeConversion  OutDataTypeStr=int16  SaturateOnIntegerOverflow=off  RndMeth=Floor
  Data Type Conversion1 : DataTypeConversion  RndMeth=Simplest  SaturateOnIntegerOverflow=off
  Delay : Delay  DelayLength=1
  Subsystem : Subsystem
  theta_e : Outport  InitialOutput=0
  wires:
  Data Type Conversion1/1 -> Add1/2
  Data Type Conversion/1 -> Data Type Conversion1/1
  Add/1 -> Data Type Conversion/1, Add1/1
  Add1/1 -> theta_e/1
  Theta_e_prev/1 -> Add/2
  Constant/1 -> Delay/1
  Delay/1 -> Subsystem/Enable
  Theta/1 -> Subsystem/1(Input)
  Subsystem/1(Out1) -> Add/1

== system mcb_pmsm_foc_sensorless_f28069MLaunchPad/Current Control/Input Scaling/Calculate position and speed/Extended EMF Observer ==
  InputSignals : Inport
  Action Port : ActionPort  ActionPortLabel=case [ 2 ]:
  Data Store Read1 : DataStoreRead  DataStoreName=Enable  IndexOptions=Index vector (dialog)  Indices=1  OutputSizes=1
  Demux1 : Demux
  Extended EMF Observer : mcbsensorlessestimatorlib/Extended EMF Observer  InputUnit=Per-unit  PosOut=Electrical position  BlkSampleTime=Ts  StatorResistance=pmsm.Rs  StatorDaxisInductance=pmsm.Ld  StatorQaxisInductance=pmsm.Lq  MaxApplicationSpeed=pmsm.N_base  PolePairs=pmsm.p  MaxStatorVoltage=PU_System.V_base  MaxStatorCurrent=PU_System.I_base  Alpha=10  EEMFCutoffFreq=7500  Kp=250  Ki=200000  N_points=1024  SpeedCutoffFreq=15  PositionUnit=Per-unit  PositionDataType=dataType  SpeedUnit=Per-unit  PerUnitSpeed=PU_System.N_base  SpeedDataType=dataType  TableDatatype=single
      settings: LibrarySourceBlock=mcblib/Sensorless Estimators/Extended EMF Observer
  Logical Operator : Logic  Operator=NOT  IconShape=distinctive  AllPortsSameDT=off  OutDataTypeStr=boolean
  Mux2 : Mux  Inputs=2
  Position/Speed : Outport
  wires:
  Mux2/1 -> Position/Speed/1
  Demux1/3 -> Extended EMF Observer/3  "Ialpha"
  Demux1/4 -> Extended EMF Observer/4  "Ibeta"
  Logical Operator/1 -> Extended EMF Observer/5
  Data Store Read1/1 -> Logical Operator/1
  Demux1/1 -> Extended EMF Observer/1
  Demux1/2 -> Extended EMF Observer/2
  InputSignals/1 -> Demux1/1
  Extended EMF Observer/1 -> Mux2/1
  Extended EMF Observer/2 -> Mux2/2

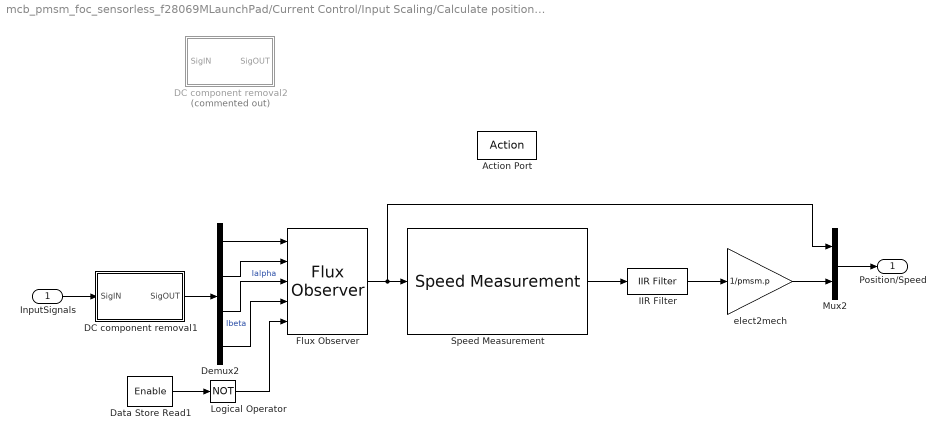
== system mcb_pmsm_foc_sensorless_f28069MLaunchPad/Current Control/Input Scaling/Calculate position and speed/Flux Observer ==
  InputSignals : Inport
  Action Port : ActionPort  ActionPortLabel=case [ 1 ]:
  DC component removal1 : Subsystem
  DC component removal2 : Subsystem  Commented=on
  Data Store Read1 : DataStoreRead  DataStoreName=Enable  IndexOptions=Index vector (dialog)  Indices=1  OutputSizes=1
  Demux2 : Demux
  Flux Observer : mcbpositiondecoderlib/Flux Observer  MotorSelection=PMSM  DataTypeSelect=off  BlockInputUnit=Per-unit  PerUnitVoltage=PU_System.V_base  PerUnitCurrent=PU_System.I_base  PositionSelect=on  FluxSelect=off  TorqueSelect=off  PolePairs=4  StatorResistance=pmsm.Rs  StatorDAxisInductance=pmsm.Ld  StatorLeakageInductance=0.0068  RotorLeakageInductance=0.0068  MagnetizingInductance=0.0300  CutoffFreq=3.1863  BlockSampleTime=Ts  ParameterBusInput=off  PositionUnit=Per-unit  PositionDatatype=dataType  FluxUnit=Weber  PerUnitFlux=0.1  FluxDatatype=single  TorqueUnit=Nm  PerUnitTorque=100  TorqueDatatype=single  DataType=0
  IIR Filter : mcbcontrolslib/IIR Filter  VariantControl=Low Pass Filter  VariantSelect=Low-pass  FilterConstantInputType=Specify via dialog  Filter_constant=0.01  advancedSettings=off  Ts=50e-6  cutOff_freq=32.1525
  Logical Operator : Logic  Operator=NOT  IconShape=distinctive  AllPortsSameDT=off  OutDataTypeStr=boolean
  Mux2 : Mux  Inputs=2
  Speed Measurement : mcbpositiondecoderlib/Speed Measurement  PositionUnit=Per unit  PositionScalingDatatype=uint32  SpeedCalculationMode=Time interval for speed calculation  SampleTimeAsync=Ts  MaximumApplicationSpeed=60000  SpeedResolution=5e-6  DelayLength=10  MaximumMeasurableSpeed=-0.96703  MeasurableSpeedResolution=1.5351e-11  SpeedUnit=Per unit based on dialog  PerUnitSpeed=PU_System.N_base  SpeedDataType=dataType
  elect2mech : Gain  Gain=1/pmsm.p  RndMeth=Simplest  OutDataTypeStr=Inherit: Same as input
  Position/Speed : Outport
  wires:
  InputSignals/1 -> DC component removal1/1(SigIN)
  Demux2/1 -> Flux Observer/1
  Demux2/2 -> Flux Observer/2
  Mux2/1 -> Position/Speed/1
  Speed Measurement/1 -> IIR Filter/1
  elect2mech/1 -> Mux2/2
  Demux2/3 -> Flux Observer/3  "Ialpha"
  Demux2/4 -> Flux Observer/4  "Ibeta"
  IIR Filter/1 -> elect2mech/1
  Flux Observer/1 -> Mux2/1, Speed Measurement/1
  Logical Operator/1 -> Flux Observer/5
  Data Store Read1/1 -> Logical Operator/1
  DC component removal1/1(SigOUT) -> Demux2/1

== system mcb_pmsm_foc_sensorless_f28069MLaunchPad/Current Control/Input Scaling/Calculate position and speed/Sliding Mode Observer ==
  InputSignals : Inport
  Action Port : ActionPort  ActionPortLabel=case [ 0 ]:
  Data Store Read1 : DataStoreRead  DataStoreName=Enable  IndexOptions=Index vector (dialog)  Indices=1  OutputSizes=1
  Demux1 : Demux
  Logical Operator : Logic  Operator=NOT  IconShape=distinctive  AllPortsSameDT=off  OutDataTypeStr=boolean
  Mux : Mux  Inputs=2
  Sliding Mode Observer1 : mcbsensorlessestimatorlib/Sliding Mode Observer  InputUnit=Per-unit  BlkSampleTime=Ts  StatorResistance=pmsm.Rs  StatorInductance=pmsm.Ld  MaxApplicationSpeed=pmsm.N_base  PolePairs=pmsm.p  MaxStatorVoltage=PU_System.V_base  MaxStatorCurrent=PU_System.I_base  DisturbanceObserverGain=smo.BackEmfObsGain  CurrentObserverGain=smo.CurrentObsGain  CutoffFreq=smo.CutoffFreq  PositionUnit=Per unit  PositionDataType=dataType  SpeedUnit=Per unit  PerUnitSpeed=PU_System.N_base  SpeedDataType=dataType
  Position/Speed : Outport
  wires:
  Mux/1 -> Position/Speed/1
  Demux1/1 -> Sliding Mode Observer1/1
  Demux1/2 -> Sliding Mode Observer1/2
  Demux1/4 -> Sliding Mode Observer1/4  "Ibeta"
  Demux1/3 -> Sliding Mode Observer1/3  "Ialpha"
  Sliding Mode Observer1/1 -> Mux/1
  Sliding Mode Observer1/2 -> Mux/2
  InputSignals/1 -> Demux1/1
  Data Store Read1/1 -> Logical Operator/1
  Logical Operator/1 -> Sliding Mode Observer1/5

== system mcb_pmsm_foc_sensorless_f28069MLaunchPad/Current Control/SCI_Tx/Code Generation/CodeGeneration ==
  Input : Inport
  Add : Sum  Inputs=+-  OutDataTypeStr=Inherit: Same as first input
  Demux2 : Demux  Outputs=2
  Index Vector : MultiPortSwitch  Inputs=1  SaturateOnIntegerOverflow=off  InputSameDT=off
  SCI Transmit : c280xlib/SCI Transmit  sciModule=A  dataHead=''  dataTail=''  frameSize=1  blockingMode=on  outputStatus=off
  While Iterator : WhileIterator  MaxIters=-1  WhileBlockType=do-while  ShowIterationPort=on  OutputDataType=int16
  wires:
  While Iterator/1 -> Add/2, Index Vector/1
  Demux2/1 -> Index Vector/2
  Index Vector/1 -> SCI Transmit/1
  Add/1 -> While Iterator/1
  Demux2/2 -> Add/1
  Input/1 -> Demux2/1

== system mcb_pmsm_foc_sensorless_f28069MLaunchPad/Hardware Init/Variant Subsystem/Code Generation/Calculate ADC Offset  ==
  Enable : EnablePort
  Constant : Constant  Value=8
  Constant1 : Constant  Value=inverter.CtSensOffsetMax  OutDataTypeStr=Inherit: Inherit via back propagation
  Constant2 : Constant  Value=inverter.CtSensOffsetMin  OutDataTypeStr=Inherit: Inherit via back propagation
  Divide : Product  Inputs=*/  OutDataTypeStr=uint16
  Divide1 : Product  Inputs=*/  OutDataTypeStr=uint16
  For Iterator Subsystem : Subsystem  TreatAsAtomicUnit=on
  If : If  NumInputs=3  IfExpression=u1 > u3 & u1 < u2
  If Action Subsystem : Subsystem  TreatAsAtomicUnit=on
  If Action Subsystem1 : Subsystem  TreatAsAtomicUnit=on
  If Action Subsystem2 : Subsystem  TreatAsAtomicUnit=on
  If Action Subsystem3 : Subsystem  TreatAsAtomicUnit=on
  If1 : If  NumInputs=3  IfExpression=u1 > u3 & u1 < u2
  wires:
  For Iterator Subsystem/2(Out2) -> Divide1/1
  Divide/1 -> If Action Subsystem/1(In1), If/1
  For Iterator Subsystem/1(Out1) -> Divide/1
  Constant/1 -> Divide/2, Divide1/2
  Divide1/1 -> If1/1, If Action Subsystem2/1(In1)
  If/1 -> If Action Subsystem/Action
  If/2 -> If Action Subsystem1/Action
  If1/1 -> If Action Subsystem2/Action
  If1/2 -> If Action Subsystem3/Action
  Constant1/1 -> If1/2, If/2
  Constant2/1 -> If/3, If1/3

== system mcb_pmsm_foc_sensorless_f28069MLaunchPad/Hardware Init/Variant Subsystem/Code Generation/DRV Enable ==
  In : Inport
  DRV830x_Enable : Constant  OutDataTypeStr=Inherit: Inherit via back propagation
  Demux : Demux  Outputs=2
  Digital Output : c2806xlib/Digital Output  GPIO_Number=GPIO50~GPIO55  GPIO_Bit0=off  GPIO_BIT0_Toggle=off  GPIO_Bit1=off  GPIO_BIT1_Toggle=off  GPIO_Bit2=on  GPIO_BIT2_Toggle=off  GPIO_Bit3=off  GPIO_BIT3_Toggle=off  GPIO_Bit4=off  GPIO_BIT4_Toggle=off  GPIO_Bit5=off  GPIO_BIT5_Toggle=off  GPIO_Bit6=off  GPIO_BIT6_Toggle=off  GPIO_Bit7=off  GPIO_BIT7_Toggle=off
  Display : Display
      settings: Format=hex (Stored Integer)
  Display1 : Display
      settings: Format=hex (Stored Integer)
  SPI Master Transfer : c280xlib/SPI Controller Transfer  SPISelect=SPI_A  ClockPolarity=Rising_edge  ClockPhase=No_delay  SPIModule=uint32(0)  Mode=Master  BusSpeed=uint32(1000000)  FirstBitToTransfer=Most significant bit (MSB)  ClockMode=0  BlockFunction=Transfer  EnableRegisterAddress=off  RegisterAddress=0  OutputDataType=int8  OutputDataLength=1  DataBits=16  UseCustomSSPin=Provided by the SPI peripheral  ActiveLowSSPin=Active low  Pin=61
  SPI Master Transfer1 : c280xlib/SPI Controller Transfer  SPISelect=SPI_A  ClockPolarity=Rising_edge  ClockPhase=No_delay  SPIModule=uint32(0)  Mode=Master  BusSpeed=uint32(1000000)  FirstBitToTransfer=Most significant bit (MSB)  ClockMode=0  BlockFunction=Transfer  EnableRegisterAddress=off  RegisterAddress=0  OutputDataType=int8  OutputDataLength=1  DataBits=16  UseCustomSSPin=Provided by the SPI peripheral  ActiveLowSSPin=Active low  Pin=61
  wires:
  Demux/2 -> SPI Master Transfer1/1
  SPI Master Transfer1/1 -> Display1/1
  SPI Master Transfer/1 -> Display/1
  Demux/1 -> SPI Master Transfer/1
  In/1 -> Demux/1
  DRV830x_Enable/1 -> Digital Output/1

== system mcb_pmsm_foc_sensorless_f28069MLaunchPad/Hardware Init/Variant Subsystem/Code Generation/Default ADC Offset ==
  Enable : EnablePort
  Constant : Constant  Value=inverter.CtSensAOffset  OutDataTypeStr=Inherit: Inherit via back propagation
  Constant1 : Constant  Value=inverter.CtSensBOffset  OutDataTypeStr=Inherit: Inherit via back propagation
  Data Store Write1 : DataStoreWrite  DataStoreName=IaOffset  IndexOptions=Index vector (dialog)  Indices=1  OutputSizes=1
  Data Store Write2 : DataStoreWrite  DataStoreName=IbOffset  IndexOptions=Index vector (dialog)  Indices=1  OutputSizes=1
  wires:
  Constant/1 -> Data Store Write1/1
  Constant1/1 -> Data Store Write2/1

== system mcb_pmsm_foc_sensorless_f28069MLaunchPad/Current Control/Closed Loop/Open_Loop_Control/Accumulate1/Subsystem ==
  Input : Inport
  Enable : EnablePort
  Out1 : Outport  InitialOutput=0
  wires:
  Input/1 -> Out1/1

== system mcb_pmsm_foc_sensorless_f28069MLaunchPad/Current Control/Input Scaling/Calculate position and speed/Flux Observer/DC component removal1 ==
  SigIN : Inport
  IIR Filter : mcbcontrolslib/IIR Filter  VariantControl=Low Pass Filter  VariantSelect=High-pass  FilterConstantInputType=Specify via dialog  Filter_constant=0.0005*(Ts/50e-6)  advancedSettings=on  Ts=50e-6  cutOff_freq=1
  SigOUT : Outport
  wires:
  SigIN/1 -> IIR Filter/1
  IIR Filter/1 -> SigOUT/1

== system mcb_pmsm_foc_sensorless_f28069MLaunchPad/Current Control/Input Scaling/Calculate position and speed/Flux Observer/DC component removal2 ==
  SigIN : Inport
  IIR Filter : mcbcontrolslib/IIR Filter  VariantControl=Low Pass Filter  VariantSelect=Low-pass  FilterConstantInputType=Specify via dialog  Filter_constant=0.005*(Ts/50e-6)  advancedSettings=off  Ts=50e-6  cutOff_freq=1
  Sum6 : Sum  Inputs=|+-  RndMeth=Simplest  OutDataTypeStr=Inherit: Same as first input
  SigOUT : Outport
  wires:
  Sum6/1 -> SigOUT/1
  SigIN/1 -> Sum6/1, IIR Filter/1
  IIR Filter/1 -> Sum6/2

== system mcb_pmsm_foc_sensorless_f28069MLaunchPad/Hardware Init/Variant Subsystem/Code Generation/Calculate ADC Offset /For Iterator Subsystem ==
  Demux : Demux  Outputs=2
  For Iterator : ForIterator  IterationLimit=16  IterationVariableDataType=uint16
  IA/IB Measurement : c2802xlib/ADC  blkParamProc=C2000  ADCModule=1  samplingMode=Simultaneous sample mode  ADCResolution=12-bit (Single-ended input)  useSOC1=SOC0  useSOC2=SOC2_SOC3  SOCAcquisitionWindow=7  SOCTriggerSource=Software  SOCInterruptTrigger=No ADCINT  Ts=-1  dType=uint16  postInterrupt=off  interruptSel=ADCINT1  ADCINTContinuous=on  endma=off  chdma=1  conv1=ADCINA0  conv2=ADCINA0 and ADCINB0  conv1_Type4=ADCIN0  conv2_Type4=ADCIN0 and ADCIN1
  If : If  IfExpression=u1 > 8  ShowElse=off
  If Action Subsystem : Subsystem  TreatAsAtomicUnit=on
  Out1 : Outport
  Out2 : Outport  Port=2
  wires:
  For Iterator/1 -> If/1
  If Action Subsystem/1(Out1) -> Out1/1
  If Action Subsystem/2(Out2) -> Out2/1
  If/1 -> If Action Subsystem/Action
  Demux/1 -> If Action Subsystem/1(In1)
  Demux/2 -> If Action Subsystem/2(In2)
  IA/IB Measurement/1 -> Demux/1

== system mcb_pmsm_foc_sensorless_f28069MLaunchPad/Hardware Init/Variant Subsystem/Code Generation/Calculate ADC Offset /If Action Subsystem ==
  In1 : Inport
  Action Port : ActionPort
  Data Store Write1 : DataStoreWrite  DataStoreName=IaOffset  IndexOptions=Index vector (dialog)  Indices=1  OutputSizes=1
  wires:
  In1/1 -> Data Store Write1/1

== system mcb_pmsm_foc_sensorless_f28069MLaunchPad/Hardware Init/Variant Subsystem/Code Generation/Calculate ADC Offset /If Action Subsystem1 ==
  Action Port : ActionPort
  Constant : Constant  Value=inverter.CtSensAOffset  OutDataTypeStr=Inherit: Inherit via back propagation
  Data Store Write1 : DataStoreWrite  DataStoreName=IaOffset  IndexOptions=Index vector (dialog)  Indices=1  OutputSizes=1
  wires:
  Constant/1 -> Data Store Write1/1

== system mcb_pmsm_foc_sensorless_f28069MLaunchPad/Hardware Init/Variant Subsystem/Code Generation/Calculate ADC Offset /If Action Subsystem2 ==
  In1 : Inport
  Action Port : ActionPort
  Data Store Write2 : DataStoreWrite  DataStoreName=IbOffset  IndexOptions=Index vector (dialog)  Indices=1  OutputSizes=1
  wires:
  In1/1 -> Data Store Write2/1

== system mcb_pmsm_foc_sensorless_f28069MLaunchPad/Hardware Init/Variant Subsystem/Code Generation/Calculate ADC Offset /If Action Subsystem3 ==
  Action Port : ActionPort
  Constant1 : Constant  Value=inverter.CtSensBOffset  OutDataTypeStr=Inherit: Inherit via back propagation
  Data Store Write2 : DataStoreWrite  DataStoreName=IbOffset  IndexOptions=Index vector (dialog)  Indices=1  OutputSizes=1
  wires:
  Constant1/1 -> Data Store Write2/1
